simulink model "sm_pump_triplex"  (R2025a)
settings: Solver=VariableStepAuto  StartTime=0.0  StopTime=1.5  RelTol=1e-3  EnableMultiTasking=on
undefined symbols (not defined in the file): pOut_Init_WKSP, smiData, TRP_Par, X, Y, Z
libraries: sm_lib x43, fl_lib x30, nesl_utility x11, simulink x10, SimscapeFluids_lib x3, sm_pump_triplex_lib x3, ee_lib x2, Multibody_Multiphysics_Lib x1
(part 2 of 3)

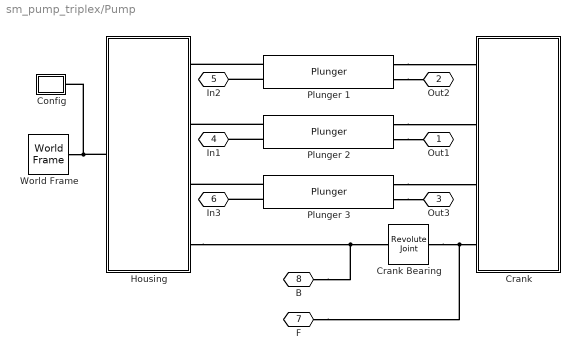
== system sm_pump_triplex/Pump ==
  Config : Subsystem
  Crank : Subsystem  mask(Crankshaft){shaft_len=shaft_len_P, shaft_rad=shaft_rad_P, web_rad=web_rad_P, web_len=web_len_P, motor_shaft_rad=motor_shaft_rad_P, motor_shaft_len=motor_shaft_len_P, shaft_pos=shaft_pos_P, crank_rho=crank_rho_P, motor_shaft_clr=motor_shaft_clr_P, crank_clr=crank_clr_P, crank_opc=crank_opc_P}
      mask prompts: shaft_pos "Crankpin Axis Offset (m)"; crank_rho "Density (kg/m^3)"; motor_shaft_clr "Motor Shaft Color [RGB]"; crank_clr "Crank Color [RGB]"; crank_opc "Opacity (0-1)"
      mask help: Models pump crankshaft with three crankpins, each offset by 120 degrees from the crankshaft axis.
      mask DialogControl text_radius Prompt: Radius (m)
      mask DialogControl text_length Prompt: Length (m)
      mask DialogControl text_crankpin Prompt: Crankpin
      mask DialogControl text_web Prompt: Web
      mask DialogControl text_motor_shaft Prompt: Motor Shaft
      mask DialogControl cont_crank_vis Prompt: Crankshaft Visualization
      mask Display: image('sm_pump_triplex_Crank_IMAGE.png');
  Crank Bearing : sm_lib/Joints/Revolute Joint  JointMode=Normal  CompositeWrenchDir=FollowerOnBase  CompositeWrenchFrame=BaseFrame  SenseConstraintForce=off  SenseConstraintTorque=off  SenseTotalForce=off  SenseTotalTorque=off  PositionTargetSpecify=off  PositionTargetPriority=High  PositionTargetValue=0  PositionTargetValueUnits=deg  VelocityTargetSpecify=off  VelocityTargetPriority=High  VelocityTargetValue=0  VelocityTargetValueUnits=deg/s  EquilibriumPosition=0  EquilibriumPositionUnits=deg  SpringStiffness=0  SpringStiffnessUnits=N*m/deg  DampingCoefficient=bearing_visc_frict  DampingCoefficientUnits=N*m/(deg/s)  LowerLimitSpecify=off  LowerLimitBound=-90  LowerLimitBoundUnits=deg  LowerLimitStiffness=1e4  LowerLimitStiffnessUnits=N*m/deg  LowerLimitDamping=10  LowerLimitDampingUnits=N*m/(deg/s)  LowerLimitTransitionRegionWidth=0.1  LowerLimitTransitionRegionWidthUnits=deg  UpperLimitSpecify=off  UpperLimitBound=90  UpperLimitBoundUnits=deg  UpperLimitStiffness=1e4  UpperLimitStiffnessUnits=N*m/deg  UpperLimitDamping=10  UpperLimitDampingUnits=N*m/(deg/s)  UpperLimitTransitionRegionWidth=0.1  UpperLimitTransitionRegionWidthUnits=deg  TorqueActuationMode=NoTorque  MotionActuationMode=ComputedMotion  SensePosition=off  SenseVelocity=off  SenseAcceleration=off  SenseTorqueForce=off  SenseLowerLimitTorqueForce=off  SenseUpperLimitTorqueForce=off
  Housing : Subsystem
      mask Display: image('sm_pump_triplex_Housing_IMAGE.png');
  Plunger 1 : sm_pump_triplex_lib/Plunger  cyl_gap=cyl_gap_P  cyl_rad_out=cyl_rad_out_P  cyl_len=cyl_len_P  cyl_stroke=cyl_stroke_P  cyl_rad_in=0  cyl_xc_rev=0  cyl_frict_brkway_frc=cyl_frict_brkway_frc_P  cyl_frict_brkway_vel=cyl_frict_brkway_vel_P  cyl_frict_col_frc=cyl_frict_col_frc_P  cyl_frict_visc_coef=cyl_frict_visc_coef_P  cyl_rho=cyl_rho_P  cyl_clr=cyl_clr_P  cyl_opc=cyl_opc_P  plgB_len=plgB_len_P  plgB_rad=plgB_rad_P  stem_len=stem_len_P  stem_rad=stem_rad_P  pin_len=pin_len_P  pin_rad=pin_rad_P  cup_rad_out=cup_rad_out_P  cup_thk=cup_thk_P  cup_len=cup_len_P  cup_pinOffset=cup_pinOffset_P  cup_rad_in=0  plg_rho=plg_rho_P  plg_clr=plg_clr_P  plg_opc=plg_opc_P  conrod_len=conrod_len_P  conrod_web_widP=conrod_web_widP_P  conrod_web_widC=conrod_web_widC_P  conrod_web_offC=0  conrod_web_offP=0  conrod_web_len=0  conrod_web_xc=0  conrod_ringC_wid=conrod_ringC_wid_P  conrod_ringP_wid=conrod_ringP_wid_P  crank_shaft_rad=crank_shaft_rad_P  conrod_ringC_or=0  conrod_ringP_or=0  conrod_ringC_xc_rev=0  conrod_ringP_xc_rev=0  conrod_thk=conrod_thk_P  conrod_rho=conrod_rho_P  conrod_clr=conrod_clr_P  conrod_opc=conrod_opc_P  chkv_in_maxA=chkv_in_maxA_P  chkv_out_maxA=chkv_out_maxA_P  chkv_press_set_popup=Set in Mask  chkv_in_crkP=chkv_in_crkP_P  chkv_out_crkP=chkv_out_crkP_P  chkv_in_maxOpenP=chkv_in_maxOpenP_P  chkv_out_maxOpenP=chkv_out_maxOpenP_P  chkv_vis_popup=On  chkv_vis_rad_in=chkv_vis_rad_in_P  chkv_vis_rad_out=chkv_vis_rad_out_P  chkv_vis_clr_in=chkv_vis_clr_in_P  chkv_vis_clr_out=chkv_vis_clr_out_P  leak_cyl_popup=Off  leak_cyl_area=leak_cyl1_area  block_in_popup=Off  block_in_factor=block_in_cyl1_factor  seal_leak_vis_len=seal_leak_vis_len_P  seal_leak_vis_rad=seal_leak_vis_rad_P  seal_leak_vis_clr=seal_leak_vis_clr_P  seal_leak_vis_opc=0  inlet_obstr_len=inlet_obstr_len_P  inlet_obstr_rad=inlet_obstr_rad_P  inlet_obstr_xc_rev=0  inlet_obstr_clr=inlet_obstr_clr_P  inlet_obstr_opc=1
  Plunger 2 : sm_pump_triplex_lib/Plunger  cyl_gap=cyl_gap_P  cyl_rad_out=cyl_rad_out_P  cyl_len=cyl_len_P  cyl_stroke=cyl_stroke_P  cyl_rad_in=0  cyl_xc_rev=0  cyl_frict_brkway_frc=cyl_frict_brkway_frc_P  cyl_frict_brkway_vel=cyl_frict_brkway_vel_P  cyl_frict_col_frc=cyl_frict_col_frc_P  cyl_frict_visc_coef=cyl_frict_visc_coef_P  cyl_rho=cyl_rho_P  cyl_clr=cyl_clr_P  cyl_opc=cyl_opc_P  plgB_len=plgB_len_P  plgB_rad=plgB_rad_P  stem_len=stem_len_P  stem_rad=stem_rad_P  pin_len=pin_len_P  pin_rad=pin_rad_P  cup_rad_out=cup_rad_out_P  cup_thk=cup_thk_P  cup_len=cup_len_P  cup_pinOffset=cup_pinOffset_P  cup_rad_in=0  plg_rho=plg_rho_P  plg_clr=plg_clr_P  plg_opc=plg_opc_P  conrod_len=conrod_len_P  conrod_web_widP=conrod_web_widP_P  conrod_web_widC=conrod_web_widC_P  conrod_web_offC=0  conrod_web_offP=0  conrod_web_len=0  conrod_web_xc=0  conrod_ringC_wid=conrod_ringC_wid_P  conrod_ringP_wid=conrod_ringP_wid_P  crank_shaft_rad=crank_shaft_rad_P  conrod_ringC_or=0  conrod_ringP_or=0  conrod_ringC_xc_rev=0  conrod_ringP_xc_rev=0  conrod_thk=conrod_thk_P  conrod_rho=conrod_rho_P  conrod_clr=conrod_clr_P  conrod_opc=conrod_opc_P  chkv_in_maxA=chkv_in_maxA_P  chkv_out_maxA=chkv_out_maxA_P  chkv_press_set_popup=Set in Mask  chkv_in_crkP=chkv_in_crkP_P  chkv_out_crkP=chkv_out_crkP_P  chkv_in_maxOpenP=chkv_in_maxOpenP_P  chkv_out_maxOpenP=chkv_out_maxOpenP_P  chkv_vis_popup=On  chkv_vis_rad_in=chkv_vis_rad_in_P  chkv_vis_rad_out=chkv_vis_rad_out_P  chkv_vis_clr_in=chkv_vis_clr_in_P  chkv_vis_clr_out=chkv_vis_clr_out_P  leak_cyl_popup=Off  leak_cyl_area=leak_cyl2_area  block_in_popup=Off  block_in_factor=block_in_cyl2_factor  seal_leak_vis_len=seal_leak_vis_len_P  seal_leak_vis_rad=seal_leak_vis_rad_P  seal_leak_vis_clr=seal_leak_vis_clr_P  seal_leak_vis_opc=0  inlet_obstr_len=inlet_obstr_len_P  inlet_obstr_rad=inlet_obstr_rad_P  inlet_obstr_xc_rev=0  inlet_obstr_clr=inlet_obstr_clr_P  inlet_obstr_opc=1
  Plunger 3 : sm_pump_triplex_lib/Plunger  cyl_gap=cyl_gap_P  cyl_rad_out=cyl_rad_out_P  cyl_len=cyl_len_P  cyl_stroke=cyl_stroke_P  cyl_rad_in=0  cyl_xc_rev=0  cyl_frict_brkway_frc=cyl_frict_brkway_frc_P  cyl_frict_brkway_vel=cyl_frict_brkway_vel_P  cyl_frict_col_frc=cyl_frict_col_frc_P  cyl_frict_visc_coef=cyl_frict_visc_coef_P  cyl_rho=cyl_rho_P  cyl_clr=cyl_clr_P  cyl_opc=cyl_opc_P  plgB_len=plgB_len_P  plgB_rad=plgB_rad_P  stem_len=stem_len_P  stem_rad=stem_rad_P  pin_len=pin_len_P  pin_rad=pin_rad_P  cup_rad_out=cup_rad_out_P  cup_thk=cup_thk_P  cup_len=cup_len_P  cup_pinOffset=cup_pinOffset_P  cup_rad_in=0  plg_rho=plg_rho_P  plg_clr=plg_clr_P  plg_opc=plg_opc_P  conrod_len=conrod_len_P  conrod_web_widP=conrod_web_widP_P  conrod_web_widC=conrod_web_widC_P  conrod_web_offC=0  conrod_web_offP=0  conrod_web_len=0  conrod_web_xc=0  conrod_ringC_wid=conrod_ringC_wid_P  conrod_ringP_wid=conrod_ringP_wid_P  crank_shaft_rad=crank_shaft_rad_P  conrod_ringC_or=0  conrod_ringP_or=0  conrod_ringC_xc_rev=0  conrod_ringP_xc_rev=0  conrod_thk=conrod_thk_P  conrod_rho=conrod_rho_P  conrod_clr=conrod_clr_P  conrod_opc=conrod_opc_P  chkv_in_maxA=chkv_in_maxA_P  chkv_out_maxA=chkv_out_maxA_P  chkv_press_set_popup=Set in Mask  chkv_in_crkP=chkv_in_crkP_P  chkv_out_crkP=chkv_out_crkP_P  chkv_in_maxOpenP=chkv_in_maxOpenP_P  chkv_out_maxOpenP=chkv_out_maxOpenP_P  chkv_vis_popup=On  chkv_vis_rad_in=chkv_vis_rad_in_P  chkv_vis_rad_out=chkv_vis_rad_out_P  chkv_vis_clr_in=chkv_vis_clr_in_P  chkv_vis_clr_out=chkv_vis_clr_out_P  leak_cyl_popup=Off  leak_cyl_area=leak_cyl3_area  block_in_popup=Off  block_in_factor=block_in_cyl3_factor  seal_leak_vis_len=seal_leak_vis_len_P  seal_leak_vis_rad=seal_leak_vis_rad_P  seal_leak_vis_clr=seal_leak_vis_clr_P  seal_leak_vis_opc=0  inlet_obstr_len=inlet_obstr_len_P  inlet_obstr_rad=inlet_obstr_rad_P  inlet_obstr_xc_rev=0  inlet_obstr_clr=inlet_obstr_clr_P  inlet_obstr_opc=1
  World Frame : sm_lib/Frames and Transforms/World Frame
  Out1 : PMIOPort  Side=Right
  Out2 : PMIOPort  Port=2  Side=Right
  Out3 : PMIOPort  Port=3  Side=Right
  In1 : PMIOPort  Port=4  Side=Right
  In2 : PMIOPort  Port=5  Side=Right
  In3 : PMIOPort  Port=6  Side=Right
  F : PMIOPort  Port=7  Side=Left
  B : PMIOPort  Port=8  Side=Left
  connections:
  Housing/LConn1 -- World Frame/RConn1 -- Config/RConn1
  Plunger 2/LConn1 -- Housing/RConn2
  Plunger 1/LConn2 -- In2/RConn1
  Plunger 1/RConn1 -- Crank/LConn1
  Plunger 2/RConn1 -- Crank/LConn2
  Plunger 3/LConn2 -- In3/RConn1
  Plunger 3/RConn2 -- Out3/RConn1
  Plunger 1/LConn1 -- Housing/RConn1
  Plunger 2/LConn2 -- In1/RConn1
  Plunger 3/LConn1 -- Housing/RConn3
  Housing/RConn4 -- B/RConn1 -- Crank Bearing/LConn1
  Crank Bearing/RConn1 -- F/RConn1 -- Crank/LConn4
  Plunger 1/RConn2 -- Out2/RConn1
  Plunger 2/RConn2 -- Out1/RConn1
  Plunger 3/RConn1 -- Crank/LConn3

== system sm_pump_triplex/Sensing Current ==
  Current Sensor : fl_lib/Electrical/Electrical Sensors/Current Sensor
  Current with Noise : Scope  NumInputPorts=2
      settings: ActiveDisplayYMinimum=-5.56656  ActiveDisplayYMaximum=49.76256  DataLoggingVariableName=ScopeData2
  Measurement Noise : simulink/Sources/Band-Limited White Noise  Cov=TRP_Par.Sensors.i.Np  Ts=TRP_Par.Sensors.i.Ts  seed=[23345]
  PS-Simulink Converter : nesl_utility/PS-Simulink Converter  PhysicalDomain=network_engine_domain  SubClassName=ps_output  LeftPortType=input  RightPortType=output  PseudoPeriodic=off  Frequencies=[]  VectorFormat=1-D array  Unit=1  AffineConversion=off
  Sum1 : Sum  Inputs=++|
  Zero-Order Hold : ZeroOrderHold  SampleTime=TRP_Par.Sensors.i.Ts
  - : PMIOPort  Side=Right
  + : PMIOPort  Port=2  Side=Left
  wires:
  Measurement Noise/1 -> Sum1/1  "Noise"
  Sum1/1 -> Zero-Order Hold/1
  PS-Simulink Converter/1 -> Sum1/2, Current with Noise/2
  Zero-Order Hold/1 -> Current with Noise/1
  connections:
  PS-Simulink Converter/LConn1 -- Current Sensor/RConn1
  +/RConn1 -- Current Sensor/LConn1
  Current Sensor/RConn2 -- -/RConn1

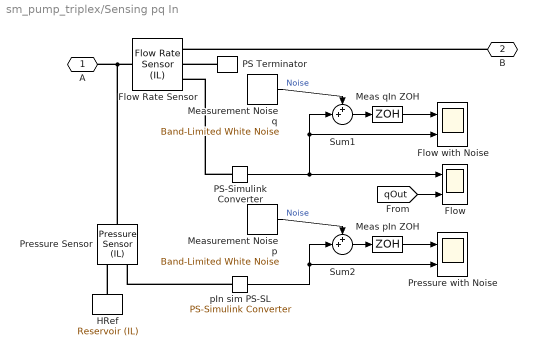
== system sm_pump_triplex/Sensing pq In ==
  Flow : Scope  NumInputPorts=2
      settings: ActiveDisplayYMinimum=-6.56594  ActiveDisplayYMaximum=59.09339  DataLoggingVariableName=ScopeData2
  Flow Rate Sensor : fl_lib/Isothermal Liquid/Sensors/Flow Rate Sensor (IL)  sensor_type=3
      settings: InternalSimscapePortConfiguration="{\"Bottom\":[],\"Left\":[{\"id\":\"A\",\"label\":\"A\",\"type\":\"foundation.isothermal_liquid.isothermal_liquid\"}],\"Right\":[{\"id\":\"B\",\"label\":\"B\",\"type\":\"foundation.isothermal_liquid.isothermal_liquid\"},{\"id\":\"M\",\"label\":\"M\",\"type\":\"output\"},{\"id\":\"V\",\"label\":\"V\",\"type\":\"output\"}],\"Top\":[]}"
      settings: LibrarySourceBlock=|
      | fl_lib/Hydraulic/Hydraulic Sensors/Hydraulic Flow Rate
      | Sensor
  Flow with Noise : Scope  NumInputPorts=2
      settings: ActiveDisplayYMinimum=-7.18648  ActiveDisplayYMaximum=60.19336
  HRef : fl_lib/Isothermal Liquid/Elements/Reservoir (IL)  reservoir_type=foundation.enum.constant_controlled.constant  pressure_spec=foundation.enum.pressure_spec.atmospheric  reservoir_pressure=0.101325 MPa
      settings: LibrarySourceBlock=fl_lib/Hydraulic/Hydraulic Elements/Hydraulic Reference
  Meas pIn ZOH : ZeroOrderHold  SampleTime=TRP_Par.Sensors.p.Ts
  Meas qIn ZOH : ZeroOrderHold  SampleTime=TRP_Par.Sensors.q.Ts
  Measurement Noise p : simulink/Sources/Band-Limited White Noise  Cov=TRP_Par.Sensors.p.Np  Ts=TRP_Par.Sensors.p.Ts  seed=[23345]
  Measurement Noise q : simulink/Sources/Band-Limited White Noise  Cov=TRP_Par.Sensors.q.Np  Ts=TRP_Par.Sensors.q.Ts  seed=[23345]
  PS Terminator : fl_lib/Physical Signals/Sinks/PS Terminator
  PS-Simulink Converter : nesl_utility/PS-Simulink Converter  PhysicalDomain=network_engine_domain  SubClassName=ps_output  LeftPortType=input  RightPortType=output  PseudoPeriodic=off  Frequencies=[]  VectorFormat=1-D array  Unit=lpm  AffineConversion=off
  Pressure Sensor : fl_lib/Isothermal Liquid/Sensors/Pressure Sensor (IL)  pressure_measure=foundation.enum.pressure_measure.difference
      settings: InternalSimscapePortConfiguration="{\"Bottom\":[],\"Left\":[{\"id\":\"A\",\"label\":\"A\",\"type\":\"foundation.isothermal_liquid.isothermal_liquid\"}],\"Right\":[{\"id\":\"B\",\"label\":\"B\",\"type\":\"foundation.isothermal_liquid.isothermal_liquid\"},{\"id\":\"P\",\"label\":\"P\",\"type\":\"output\"}],\"Top\":[]}"
      settings: LibrarySourceBlock=|
      | fl_lib/Hydraulic/Hydraulic Sensors/Hydraulic Pressure
      | Sensor
  Pressure with Noise : Scope  NumInputPorts=2
      settings: ActiveDisplayYMinimum=6.95483  ActiveDisplayYMaximum=7.36166
  Sum1 : Sum  Inputs=++|
  Sum2 : Sum  Inputs=++|
  pIn sim PS-SL : nesl_utility/PS-Simulink Converter  PhysicalDomain=network_engine_domain  SubClassName=ps_output  LeftPortType=input  RightPortType=output  PseudoPeriodic=off  Frequencies=[]  VectorFormat=1-D array  Unit=bar  AffineConversion=off
  A : PMIOPort  Side=Left
  B : PMIOPort  Port=2  Side=Right
  wires:
  Meas pIn ZOH/1 -> Pressure with Noise/1
  Measurement Noise p/1 -> Sum2/1  "Noise"
  pIn sim PS-SL/1 -> Pressure with Noise/2, Sum2/2
  Sum2/1 -> Meas pIn ZOH/1
  Meas qIn ZOH/1 -> Flow with Noise/1
  Sum1/1 -> Meas qIn ZOH/1
  Measurement Noise q/1 -> Sum1/1  "Noise"
  PS-Simulink Converter/1 -> Flow/1, Flow with Noise/2, Sum1/2
  [qOut] -> Flow/2
  connections:
  pIn sim PS-SL/LConn1 -- Pressure Sensor/RConn2
  HRef/LConn1 -- Pressure Sensor/RConn1
  Pressure Sensor/LConn1 -- Flow Rate Sensor/LConn1 -- A/RConn1
  PS Terminator/LConn1 -- Flow Rate Sensor/RConn2
  B/RConn1 -- Flow Rate Sensor/RConn1
  PS-Simulink Converter/LConn1 -- Flow Rate Sensor/RConn3

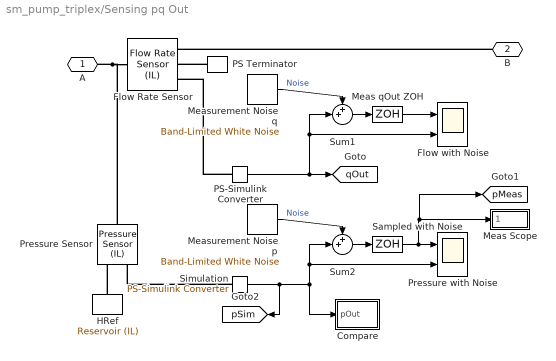
== system sm_pump_triplex/Sensing pq Out ==
  Compare : Subsystem
  Flow Rate Sensor : fl_lib/Isothermal Liquid/Sensors/Flow Rate Sensor (IL)  sensor_type=3
      settings: InternalSimscapePortConfiguration="{\"Bottom\":[],\"Left\":[{\"id\":\"A\",\"label\":\"A\",\"type\":\"foundation.isothermal_liquid.isothermal_liquid\"}],\"Right\":[{\"id\":\"B\",\"label\":\"B\",\"type\":\"foundation.isothermal_liquid.isothermal_liquid\"},{\"id\":\"M\",\"label\":\"M\",\"type\":\"output\"},{\"id\":\"V\",\"label\":\"V\",\"type\":\"output\"}],\"Top\":[]}"
      settings: LibrarySourceBlock=|
      | fl_lib/Hydraulic/Hydraulic Sensors/Hydraulic Flow Rate
      | Sensor
  Flow with Noise : Scope  NumInputPorts=2
      settings: ActiveDisplayYMinimum=-6.25341  ActiveDisplayYMaximum=51.79569
  HRef : fl_lib/Isothermal Liquid/Elements/Reservoir (IL)  reservoir_type=foundation.enum.constant_controlled.constant  pressure_spec=foundation.enum.pressure_spec.atmospheric  reservoir_pressure=0.101325 MPa
      settings: LibrarySourceBlock=fl_lib/Hydraulic/Hydraulic Elements/Hydraulic Reference
  Meas Scope : Subsystem
  Meas qOut ZOH : ZeroOrderHold  SampleTime=TRP_Par.Sensors.q.Ts
  Measurement Noise p : simulink/Sources/Band-Limited White Noise  Cov=TRP_Par.Sensors.p.Np  Ts=TRP_Par.Sensors.p.Ts  seed=[23345]
  Measurement Noise q : simulink/Sources/Band-Limited White Noise  Cov=TRP_Par.Sensors.q.Np  Ts=TRP_Par.Sensors.q.Ts  seed=[23345]
  PS Terminator : fl_lib/Physical Signals/Sinks/PS Terminator
  PS-Simulink Converter : nesl_utility/PS-Simulink Converter  PhysicalDomain=network_engine_domain  SubClassName=ps_output  LeftPortType=input  RightPortType=output  PseudoPeriodic=off  Frequencies=[]  VectorFormat=1-D array  Unit=lpm  AffineConversion=off
  Pressure Sensor : fl_lib/Isothermal Liquid/Sensors/Pressure Sensor (IL)  pressure_measure=foundation.enum.pressure_measure.difference
      settings: InternalSimscapePortConfiguration="{\"Bottom\":[],\"Left\":[{\"id\":\"A\",\"label\":\"A\",\"type\":\"foundation.isothermal_liquid.isothermal_liquid\"}],\"Right\":[{\"id\":\"B\",\"label\":\"B\",\"type\":\"foundation.isothermal_liquid.isothermal_liquid\"},{\"id\":\"P\",\"label\":\"P\",\"type\":\"output\"}],\"Top\":[]}"
      settings: LibrarySourceBlock=|
      | fl_lib/Hydraulic/Hydraulic Sensors/Hydraulic Pressure
      | Sensor
  Pressure with Noise : Scope  NumInputPorts=2
      settings: ActiveDisplayYMinimum=6.95483  ActiveDisplayYMaximum=7.36166
  Sampled with Noise : ZeroOrderHold  SampleTime=TRP_Par.Sensors.p.Ts
  Simulation : nesl_utility/PS-Simulink Converter  PhysicalDomain=network_engine_domain  SubClassName=ps_output  LeftPortType=input  RightPortType=output  PseudoPeriodic=off  Frequencies=[]  VectorFormat=1-D array  Unit=bar  AffineConversion=off
  Sum1 : Sum  Inputs=++|
  Sum2 : Sum  Inputs=++|
  A : PMIOPort  Side=Left
  B : PMIOPort  Port=2  Side=Right
  tag scope: pMeas=global, pSim=global, qOut=global
  wires:
  PS-Simulink Converter/1 -> Sum1/2, Flow with Noise/2, [qOut]
  Measurement Noise q/1 -> Sum1/1  "Noise"
  Sum1/1 -> Meas qOut ZOH/1
  Meas qOut ZOH/1 -> Flow with Noise/1
  Sum2/1 -> Sampled with Noise/1
  Simulation/1 -> [pSim], Compare/1(pOut), Sum2/2, Pressure with Noise/2
  Measurement Noise p/1 -> Sum2/1  "Noise"
  Sampled with Noise/1 -> [pMeas], Meas Scope/1(pMeas), Pressure with Noise/1
  connections:
  Pressure Sensor/LConn1 -- Flow Rate Sensor/LConn1 -- A/RConn1
  HRef/LConn1 -- Pressure Sensor/RConn1
  Simulation/LConn1 -- Pressure Sensor/RConn2
  PS Terminator/LConn1 -- Flow Rate Sensor/RConn2
  B/RConn1 -- Flow Rate Sensor/RConn1
  PS-Simulink Converter/LConn1 -- Flow Rate Sensor/RConn3

== system sm_pump_triplex/Diagnostics/Diagnostics ==
  "pOut " : Inport
  Off : Subsystem  VariantControl=Off
  On : Subsystem  VariantControl=On
  " fault" : Outport  VectorParamsAs1DForOutWhenUnconnected=off
  " hmi" : Outport  Port=2  VectorParamsAs1DForOutWhenUnconnected=off

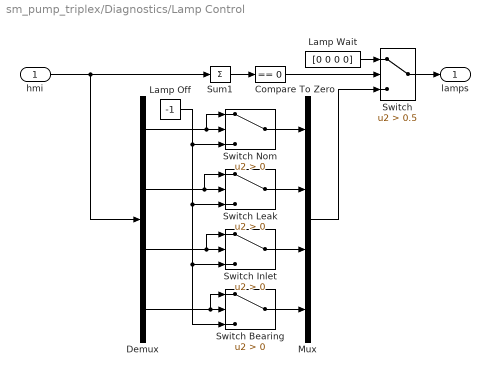
== system sm_pump_triplex/Diagnostics/Lamp Control ==
  hmi : Inport
  Compare To Zero : simulink/Logic and Bit Operations/Compare To Zero  relop===  OutDataTypeStr=boolean  ZeroCross=off
  Demux : Demux
  Lamp Off : Constant  Value=-1
  Lamp Wait : Constant  Value=[0 0 0 0]
  Mux : Mux
  Sum1 : Sum  Inputs=+
  Switch : Switch  Criteria=u2 > Threshold  Threshold=0.5  ZeroCross=off  SaturateOnIntegerOverflow=off  InputSameDT=off
  Switch Bearing : Switch  Criteria=u2 > Threshold  ZeroCross=off  SaturateOnIntegerOverflow=off  InputSameDT=off
  Switch Inlet : Switch  Criteria=u2 > Threshold  ZeroCross=off  SaturateOnIntegerOverflow=off  InputSameDT=off
  Switch Leak : Switch  Criteria=u2 > Threshold  ZeroCross=off  SaturateOnIntegerOverflow=off  InputSameDT=off
  Switch Nom : Switch  Criteria=u2 > Threshold  ZeroCross=off  SaturateOnIntegerOverflow=off  InputSameDT=off
  lamps : Outport  VectorParamsAs1DForOutWhenUnconnected=off
  wires:
  Compare To Zero/1 -> Switch/2
  Sum1/1 -> Compare To Zero/1
  hmi/1 -> Demux/1, Sum1/1
  Switch/1 -> lamps/1
  Lamp Wait/1 -> Switch/1
  Switch Nom/1 -> Mux/1
  Switch Leak/1 -> Mux/2
  Switch Inlet/1 -> Mux/3
  Switch Bearing/1 -> Mux/4
  Mux/1 -> Switch/3
  Demux/1 -> Switch Nom/1, Switch Nom/2
  Demux/2 -> Switch Leak/1, Switch Leak/2
  Demux/3 -> Switch Inlet/1, Switch Inlet/2
  Demux/4 -> Switch Bearing/1, Switch Bearing/2
  Lamp Off/1 -> Switch Bearing/3, Switch Inlet/3, Switch Leak/3, Switch Nom/3

== system sm_pump_triplex/Driver/Driver ==
  Dyno : Subsystem  VariantControl=Dyno
      mask Display: image('sm_pump_triplex_driverDyno_IMAGE.png');
  Motor : Subsystem  VariantControl=Motor  mask{winding_fault_enable=Off, winding_fault_sw=0}
      mask prompts: winding_fault_enable "Winding Fault"; winding_fault_sw "Winding Fault Input for Switch (1,2)"
      mask init:
      | if(strcmp(get_param(gcb,'winding_fault_enable'),'Off'))
      |     winding_fault_sw = 1;
      | else
      |     winding_fault_sw = 2;
      | end
      mask TypeOptions winding_fault_enable: Off | On
      mask Display:
      | image('sm_pump_triplex_driverMotor_IMAGE.png');
      | 
      | color('red');
      | if(strcmp(get_param(gcb,'winding_fault_enable'),'On'))
      |     plot([0.85 0.6],[1.1 0.9])
      |     plot([0.6 0.85],[1.1 0.9])
      | end
      | 
      | % Plot points to set plot range
      | color('white');plot(1.2,2.4);plot(-1.2,-2.4)
      | color('black');
  " F " : PMIOPort  Side=Right
  " B " : PMIOPort  Port=2  Side=Right
  " + " : PMIOPort  Port=3  Side=Left
  " - " : PMIOPort  Port=4  Side=Left

== system sm_pump_triplex/Pump/Config ==
  Mechanism Configuration : sm_lib/Utilities/Mechanism Configuration  UniformGravity=Constant  GravityVector=[0 -1 0]*9.80665  GravityVectorUnits=m/s^2  LinearizationDelta=0.001  JointModeTransitionNonlinearIterations=2
  Solver Configuration : nesl_utility/Solver Configuration  PhysicalDomain=network_engine_domain  SubClassName=solver  LeftPortType=input  RightPortType=generic  Tones=[]  Harmonics=[]  SimulateNoise=off  Profile=off  UseLocalSampling=off  EnableSwitchedLinearOptims=on  FrequencyDomain=off  UseCCode=off  RelTol=0.001  AbsTol=1e-06  MinStep=1e-09  ToWorkspace=off  RevertToSquareIcSolve=off  NumHomotopyIterations=100  PhasorMode=off  PhasorModeNumHarmonics=1  ConsistencySolver=NEWTON_FTOL  IndexReductionMethod=DerivativeReplacement  DoDC=off  ResidualTolerance=1e-10  ConsistencyTolSource=GLOBAL  ConsistencyAbsTol=0.001  ConsistencyRelTol=0.001  ConsistencyTolFactor=0.001  UseLocalSolver=off  LocalSolverChoice=NE_BACKWARD_EULER_ADVANCER  ResolveIndetEquations=on  FunctionEvalNumThread=1  LocalSolverSampleTime=0.001  DoFixedCost=off  MaxNonlinIter=3  MaxModeIter=2  ComputeImpulses=off  ImpulseIterations=2  LinearAlgebra=Sparse  LinearAlgebraNumThread=0  EquationFormulation=NE_TIME_EF  DelaysMemoryBudget=1024  AutomaticFiltering=on  FilteringTimeConstant=0.001  PartitionStorageMethod=AS_NEEDED  PartitionMemoryBudget=1024  PartitionMethod=FAST  MultibodyUseLocalSolver=off  MultibodyLocalSolverChoice=ODE1  MultibodyLocalSolverSampleTime=0.001
  C : PMIOPort  Side=Right
  connections:
  Solver Configuration/RConn1 -- C/RConn1 -- Mechanism Configuration/RConn1

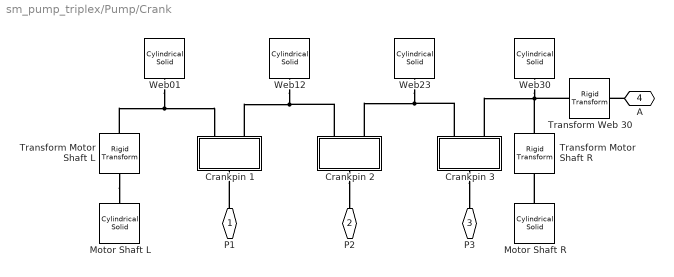
== system sm_pump_triplex/Pump/Crank ==
  Crankpin 1 : Subsystem
  Crankpin 2 : Subsystem
  Crankpin 3 : Subsystem
  Motor Shaft L : sm_lib/Body Elements/Cylindrical Solid  CylinderRadius=motor_shaft_rad  CylinderRadiusUnits=m  CylinderLength=motor_shaft_len  CylinderLengthUnits=m  ExportEntireGeometry=off  InertiaType=CalculateFromGeometry  BasedOnType=Density  Density=crank_rho  DensityUnits=kg/m^3  Mass=1  MassUnits=kg  CenterOfMass=[0 0 0]  CenterOfMassUnits=m  MomentsOfInertia=[1 1 1]  MomentsOfInertiaUnits=kg*m^2  ProductsOfInertia=[1 1 1]  ProductsOfInertiaUnits=kg*m^2  GraphicType=FromGeometry  MarkerShape=Sphere  MarkerSize=10  GraphicVisPropType=SimpleVisualProperties  GraphicDiffuseColor=motor_shaft_clr  GraphicOpacity=crank_opc  GraphicSpecularColor=[0.5 0.5 0.5 1.0]  GraphicAmbientColor=[0.15 0.15 0.15 1.0]  GraphicEmissiveColor=[0.0 0.0 0.0 1.0]  GraphicShininess=75  DoExposeReferenceFrame=on  SerializedFrames=<Frames/>
  Motor Shaft R : sm_lib/Body Elements/Cylindrical Solid  CylinderRadius=motor_shaft_rad  CylinderRadiusUnits=m  CylinderLength=motor_shaft_len  CylinderLengthUnits=m  ExportEntireGeometry=off  InertiaType=CalculateFromGeometry  BasedOnType=Density  Density=crank_rho  DensityUnits=kg/m^3  Mass=1  MassUnits=kg  CenterOfMass=[0 0 0]  CenterOfMassUnits=m  MomentsOfInertia=[1 1 1]  MomentsOfInertiaUnits=kg*m^2  ProductsOfInertia=[1 1 1]  ProductsOfInertiaUnits=kg*m^2  GraphicType=FromGeometry  MarkerShape=Sphere  MarkerSize=10  GraphicVisPropType=SimpleVisualProperties  GraphicDiffuseColor=motor_shaft_clr  GraphicOpacity=crank_opc  GraphicSpecularColor=[0.5 0.5 0.5 1.0]  GraphicAmbientColor=[0.15 0.15 0.15 1.0]  GraphicEmissiveColor=[0.0 0.0 0.0 1.0]  GraphicShininess=75  DoExposeReferenceFrame=on  SerializedFrames=<Frames/>
  Transform Motor Shaft L : sm_lib/Frames and Transforms/Rigid Transform  RotationMethod=None  FollAlignAxisA=+X  BaseAlignAxisA=+Y  FollAlignAxisB=+Y  BaseAlignAxisB=+Z  RotationStandardAxis=+Z  RotationAngle=0.0  RotationAngleUnits=deg  RotationArbitraryAxis=[0 0 1]  RotationSequenceAxes=FollowerAxes  RotationSequence=XYX  RotationSequenceAngles=[0 0 0]  RotationSequenceAnglesUnits=deg  RotationMatrix=[1 0 0; 0 1 0; 0 0 1]  Quaternion=[1 0 0 0]  TranslationMethod=StandardAxis  TranslationCartesianOffset=[0 0 0]  TranslationCartesianOffsetUnits=m  TranslationStandardAxis=+Z  TranslationStandardOffset=motor_shaft_len/2  TranslationStandardOffsetUnits=m  TranslationROffset=0  TranslationROffsetUnits=m  TranslationThetaOffset=0  TranslationThetaOffsetUnits=deg  TranslationZOffset=0  TranslationZOffsetUnits=m
  Transform Motor Shaft R : sm_lib/Frames and Transforms/Rigid Transform  RotationMethod=None  FollAlignAxisA=+X  BaseAlignAxisA=+Y  FollAlignAxisB=+Y  BaseAlignAxisB=+Z  RotationStandardAxis=+Z  RotationAngle=0.0  RotationAngleUnits=deg  RotationArbitraryAxis=[0 0 1]  RotationSequenceAxes=FollowerAxes  RotationSequence=XYX  RotationSequenceAngles=[0 0 0]  RotationSequenceAnglesUnits=deg  RotationMatrix=[1 0 0; 0 1 0; 0 0 1]  Quaternion=[1 0 0 0]  TranslationMethod=StandardAxis  TranslationCartesianOffset=[0 0 0]  TranslationCartesianOffsetUnits=m  TranslationStandardAxis=+Z  TranslationStandardOffset=motor_shaft_len/2  TranslationStandardOffsetUnits=m  TranslationROffset=0  TranslationROffsetUnits=m  TranslationThetaOffset=0  TranslationThetaOffsetUnits=deg  TranslationZOffset=0  TranslationZOffsetUnits=m
  Transform Web 30 : sm_lib/Frames and Transforms/Rigid Transform  RotationMethod=None  FollAlignAxisA=+X  BaseAlignAxisA=+Y  FollAlignAxisB=+Y  BaseAlignAxisB=+Z  RotationStandardAxis=+Z  RotationAngle=0.0  RotationAngleUnits=deg  RotationArbitraryAxis=[0 0 1]  RotationSequenceAxes=FollowerAxes  RotationSequence=XYX  RotationSequenceAngles=[0 0 0]  RotationSequenceAnglesUnits=deg  RotationMatrix=[1 0 0; 0 1 0; 0 0 1]  Quaternion=[1 0 0 0]  TranslationMethod=StandardAxis  TranslationCartesianOffset=[0 0 0]  TranslationCartesianOffsetUnits=m  TranslationStandardAxis=+Z  TranslationStandardOffset=shaft_len*1.5  TranslationStandardOffsetUnits=m  TranslationROffset=0  TranslationROffsetUnits=m  TranslationThetaOffset=0  TranslationThetaOffsetUnits=deg  TranslationZOffset=0  TranslationZOffsetUnits=m
  Web01 : sm_lib/Body Elements/Cylindrical Solid  CylinderRadius=web_rad  CylinderRadiusUnits=m  CylinderLength=web_len  CylinderLengthUnits=m  ExportEntireGeometry=off  InertiaType=CalculateFromGeometry  BasedOnType=Density  Density=crank_rho  DensityUnits=kg/m^3  Mass=1  MassUnits=kg  CenterOfMass=[0 0 0]  CenterOfMassUnits=m  MomentsOfInertia=[1 1 1]  MomentsOfInertiaUnits=kg*m^2  ProductsOfInertia=[1 1 1]  ProductsOfInertiaUnits=kg*m^2  GraphicType=FromGeometry  MarkerShape=Sphere  MarkerSize=10  GraphicVisPropType=SimpleVisualProperties  GraphicDiffuseColor=crank_clr  GraphicOpacity=crank_opc  GraphicSpecularColor=[0.5 0.5 0.5 1.0]  GraphicAmbientColor=[0.15 0.15 0.15 1.0]  GraphicEmissiveColor=[0.0 0.0 0.0 1.0]  GraphicShininess=75  DoExposeReferenceFrame=on  SerializedFrames=<Frames/>
  Web12 : sm_lib/Body Elements/Cylindrical Solid  CylinderRadius=web_rad  CylinderRadiusUnits=m  CylinderLength=web_len  CylinderLengthUnits=m  ExportEntireGeometry=off  InertiaType=CalculateFromGeometry  BasedOnType=Density  Density=crank_rho  DensityUnits=kg/m^3  Mass=1  MassUnits=kg  CenterOfMass=[0 0 0]  CenterOfMassUnits=m  MomentsOfInertia=[1 1 1]  MomentsOfInertiaUnits=kg*m^2  ProductsOfInertia=[1 1 1]  ProductsOfInertiaUnits=kg*m^2  GraphicType=FromGeometry  MarkerShape=Sphere  MarkerSize=10  GraphicVisPropType=SimpleVisualProperties  GraphicDiffuseColor=crank_clr  GraphicOpacity=crank_opc  GraphicSpecularColor=[0.5 0.5 0.5 1.0]  GraphicAmbientColor=[0.15 0.15 0.15 1.0]  GraphicEmissiveColor=[0.0 0.0 0.0 1.0]  GraphicShininess=75  DoExposeReferenceFrame=on  SerializedFrames=<Frames/>
  Web23 : sm_lib/Body Elements/Cylindrical Solid  CylinderRadius=web_rad  CylinderRadiusUnits=m  CylinderLength=web_len  CylinderLengthUnits=m  ExportEntireGeometry=off  InertiaType=CalculateFromGeometry  BasedOnType=Density  Density=crank_rho  DensityUnits=kg/m^3  Mass=1  MassUnits=kg  CenterOfMass=[0 0 0]  CenterOfMassUnits=m  MomentsOfInertia=[1 1 1]  MomentsOfInertiaUnits=kg*m^2  ProductsOfInertia=[1 1 1]  ProductsOfInertiaUnits=kg*m^2  GraphicType=FromGeometry  MarkerShape=Sphere  MarkerSize=10  GraphicVisPropType=SimpleVisualProperties  GraphicDiffuseColor=crank_clr  GraphicOpacity=crank_opc  GraphicSpecularColor=[0.5 0.5 0.5 1.0]  GraphicAmbientColor=[0.15 0.15 0.15 1.0]  GraphicEmissiveColor=[0.0 0.0 0.0 1.0]  GraphicShininess=75  DoExposeReferenceFrame=on  SerializedFrames=<Frames/>
  Web30 : sm_lib/Body Elements/Cylindrical Solid  CylinderRadius=web_rad  CylinderRadiusUnits=m  CylinderLength=web_len  CylinderLengthUnits=m  ExportEntireGeometry=off  InertiaType=CalculateFromGeometry  BasedOnType=Density  Density=crank_rho  DensityUnits=kg/m^3  Mass=1  MassUnits=kg  CenterOfMass=[0 0 0]  CenterOfMassUnits=m  MomentsOfInertia=[1 1 1]  MomentsOfInertiaUnits=kg*m^2  ProductsOfInertia=[1 1 1]  ProductsOfInertiaUnits=kg*m^2  GraphicType=FromGeometry  MarkerShape=Sphere  MarkerSize=10  GraphicVisPropType=SimpleVisualProperties  GraphicDiffuseColor=crank_clr  GraphicOpacity=crank_opc  GraphicSpecularColor=[0.5 0.5 0.5 1.0]  GraphicAmbientColor=[0.15 0.15 0.15 1.0]  GraphicEmissiveColor=[0.0 0.0 0.0 1.0]  GraphicShininess=75  DoExposeReferenceFrame=on  SerializedFrames=<Frames/>
  P1 : PMIOPort  Side=Left
  P2 : PMIOPort  Port=2  Side=Left
  P3 : PMIOPort  Port=3  Side=Left
  A : PMIOPort  Port=4  Side=Left
  connections:
  Crankpin 2/LConn2 -- Web23/RConn1 -- Crankpin 3/LConn1
  Motor Shaft R/RConn1 -- Transform Motor Shaft R/RConn1
  Crankpin 1/LConn2 -- Web12/RConn1 -- Crankpin 2/LConn1
  Crankpin 2/RConn1 -- P2/RConn1
  Web01/RConn1 -- Transform Motor Shaft L/RConn1 -- Crankpin 1/LConn1
  P1/RConn1 -- Crankpin 1/RConn1
  Crankpin 3/RConn1 -- P3/RConn1
  Transform Motor Shaft R/LConn1 -- Transform Web 30/RConn1 -- Web30/RConn1 -- Crankpin 3/LConn2
  Transform Motor Shaft L/LConn1 -- Motor Shaft L/RConn1
  A/RConn1 -- Transform Web 30/LConn1

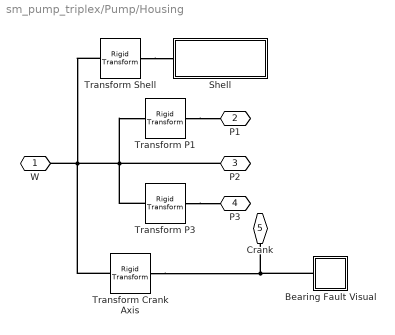
== system sm_pump_triplex/Pump/Housing ==
  Bearing Fault Visual : Subsystem
  Shell : Subsystem
  Transform Crank Axis : sm_lib/Frames and Transforms/Rigid Transform  RotationMethod=StandardAxis  FollAlignAxisA=+X  BaseAlignAxisA=+Y  FollAlignAxisB=+Y  BaseAlignAxisB=+Z  RotationStandardAxis=+Y  RotationAngle=90  RotationAngleUnits=deg  RotationArbitraryAxis=[0 0 1]  RotationSequenceAxes=FollowerAxes  RotationSequence=XYX  RotationSequenceAngles=[0 0 0]  RotationSequenceAnglesUnits=deg  RotationMatrix=[1 0 0; 0 1 0; 0 0 1]  Quaternion=[1 0 0 0]  TranslationMethod=Cartesian  TranslationCartesianOffset=crank_ax_offset  TranslationCartesianOffsetUnits=m  TranslationStandardAxis=+Z  TranslationStandardOffset=0  TranslationStandardOffsetUnits=m  TranslationROffset=0  TranslationROffsetUnits=m  TranslationThetaOffset=0  TranslationThetaOffsetUnits=deg  TranslationZOffset=0  TranslationZOffsetUnits=m
  Transform Shell : sm_lib/Frames and Transforms/Rigid Transform  RotationMethod=StandardAxis  FollAlignAxisA=+X  BaseAlignAxisA=+Y  FollAlignAxisB=+Y  BaseAlignAxisB=+Z  RotationStandardAxis=+Y  RotationAngle=180  RotationAngleUnits=deg  RotationArbitraryAxis=[0 0 1]  RotationSequenceAxes=FollowerAxes  RotationSequence=XYX  RotationSequenceAngles=[0 0 0]  RotationSequenceAnglesUnits=deg  RotationMatrix=[1 0 0; 0 1 0; 0 0 1]  Quaternion=[1 0 0 0]  TranslationMethod=Cartesian  TranslationCartesianOffset=TRP_Par.CAD.offset  TranslationCartesianOffsetUnits=m  TranslationStandardAxis=+Z  TranslationStandardOffset=0  TranslationStandardOffsetUnits=m  TranslationROffset=0  TranslationROffsetUnits=m  TranslationThetaOffset=0  TranslationThetaOffsetUnits=deg  TranslationZOffset=0  TranslationZOffsetUnits=m
  Transform P1 : sm_lib/Frames and Transforms/Rigid Transform  RotationMethod=None  FollAlignAxisA=+X  BaseAlignAxisA=+Y  FollAlignAxisB=+Y  BaseAlignAxisB=+Z  RotationStandardAxis=+Z  RotationAngle=0.0  RotationAngleUnits=deg  RotationArbitraryAxis=[0 0 1]  RotationSequenceAxes=FollowerAxes  RotationSequence=XYX  RotationSequenceAngles=[0 0 0]  RotationSequenceAnglesUnits=deg  RotationMatrix=[1 0 0; 0 1 0; 0 0 1]  Quaternion=[1 0 0 0]  TranslationMethod=StandardAxis  TranslationCartesianOffset=[0 0 0]  TranslationCartesianOffsetUnits=m  TranslationStandardAxis=+X  TranslationStandardOffset=-TRP_Par.Crank.Shaft.len  TranslationStandardOffsetUnits=m  TranslationROffset=0  TranslationROffsetUnits=m  TranslationThetaOffset=0  TranslationThetaOffsetUnits=deg  TranslationZOffset=0  TranslationZOffsetUnits=m
  Transform P3 : sm_lib/Frames and Transforms/Rigid Transform  RotationMethod=None  FollAlignAxisA=+X  BaseAlignAxisA=+Y  FollAlignAxisB=+Y  BaseAlignAxisB=+Z  RotationStandardAxis=+Z  RotationAngle=0.0  RotationAngleUnits=deg  RotationArbitraryAxis=[0 0 1]  RotationSequenceAxes=FollowerAxes  RotationSequence=XYX  RotationSequenceAngles=[0 0 0]  RotationSequenceAnglesUnits=deg  RotationMatrix=[1 0 0; 0 1 0; 0 0 1]  Quaternion=[1 0 0 0]  TranslationMethod=StandardAxis  TranslationCartesianOffset=[0 0 0]  TranslationCartesianOffsetUnits=m  TranslationStandardAxis=-X  TranslationStandardOffset=-TRP_Par.Crank.Shaft.len  TranslationStandardOffsetUnits=m  TranslationROffset=0  TranslationROffsetUnits=m  TranslationThetaOffset=0  TranslationThetaOffsetUnits=deg  TranslationZOffset=0  TranslationZOffsetUnits=m
  W : PMIOPort  Side=Left
  P1 : PMIOPort  Port=2  Side=Right
  P2 : PMIOPort  Port=3  Side=Right
  P3 : PMIOPort  Port=4  Side=Right
  Crank : PMIOPort  Port=5  Side=Right
  connections:
  Transform P3/RConn1 -- P3/RConn1
  Transform P1/RConn1 -- P1/RConn1
  Transform P3/LConn1 -- Transform Shell/LConn1 -- Transform Crank Axis/LConn1 -- W/RConn1 -- P2/RConn1 -- Transform P1/LConn1
  Transform Shell/RConn1 -- Shell/LConn1
  Transform Crank Axis/RConn1 -- Bearing Fault Visual/LConn1 -- Crank/RConn1

== system sm_pump_triplex/Sensing pq Out/Compare ==
  pOut : Inport
  Measured Data : FromWorkspace  VariableName=[pOutMeas_time pOutMeas_data]  OutputAfterFinalValue=Holding final value
  Output Pressure : Scope  NumInputPorts=2
      settings: Title=Output Pressure: Compare with Measured Data  ActiveDisplayYMinimum=6.95756  ActiveDisplayYMaximum=7.33433
  Zero-Order Hold : ZeroOrderHold  SampleTime=-1
  wires:
  pOut/1 -> Output Pressure/1  "Simulation"
  Measured Data/1 -> Zero-Order Hold/1
  Zero-Order Hold/1 -> Output Pressure/2  "Measured"

== system sm_pump_triplex/Sensing pq Out/Meas Scope ==
  pMeas : Inport
  Output Pressure Measurement : Scope
      settings: TimeSpan=1  ActiveDisplayYMinimum=6.95483  ActiveDisplayYMaximum=7.36166
  wires:
  pMeas/1 -> Output Pressure Measurement/1

== system sm_pump_triplex/Diagnostics/Diagnostics/Off ==
  pOut : Inport
  Constant : Constant  OutDataTypeStr=int8
  Constant1 : Constant  Value=[1 1 1 1]*-1
  Terminator : Terminator
  fault : Outport  VectorParamsAs1DForOutWhenUnconnected=off
  hmi : Outport  Port=2  VectorParamsAs1DForOutWhenUnconnected=off
  wires:
  Constant1/1 -> hmi/1
  Constant/1 -> fault/1
  pOut/1 -> Terminator/1

== system sm_pump_triplex/Diagnostics/Diagnostics/On ==
  pOut : Inport
  Clock : Clock
  Collect Data : MATLAB Function  TreatAsAtomicUnit=on  SystemSampleTime=TRP_Par.Sensors.q.Ts
  FFT and Classification : MATLAB Function  TreatAsAtomicUnit=on  SystemSampleTime=TRP_Par.Sensors.q.Ts*100
  Motor Speed (RPM) : Constant  Value=TRP_Par.Spec.target_spd
  Steady State : simulink/Logic and Bit Operations/Compare To Constant  relop=>=  const=time_steady_state  OutDataTypeStr=boolean  ZeroCross=off
  fault : Outport  VectorParamsAs1DForOutWhenUnconnected=off
  hmi : Outport  Port=2  VectorParamsAs1DForOutWhenUnconnected=off
  wires:
  Clock/1 -> Steady State/1
  Steady State/1 -> FFT and Classification/2(enablePred)
  FFT and Classification/1(faultState) -> fault/1
  Motor Speed (RPM)/1 -> FFT and Classification/3(cmdSpeed)
  Collect Data/1(pArray) -> FFT and Classification/1(pArray)
  pOut/1 -> Collect Data/1(pOut)
  FFT and Classification/2(hmiVec) -> hmi/1

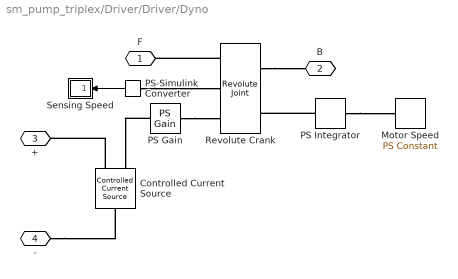
== system sm_pump_triplex/Driver/Driver/Dyno ==
  Controlled Current Source : fl_lib/Electrical/Electrical Sources/Controlled Current Source
  Motor Speed : fl_lib/Physical Signals/Sources/PS Constant  constant=TRP_Par.Spec.target_spd*2*pi/60 rad/s
  PS Gain : fl_lib/Physical Signals/Functions/PS Gain  gain=1 A/(N*m)
  PS Integrator : fl_lib/Physical Signals/Linear Operators/PS Integrator  reset_method=foundation.enum.IntegratorResetSpec.None  initial_condition_spec=foundation.enum.IntegratorICSpec.Internal  saturation_spec=foundation.enum.IntegratorSaturationSpec.None  saturation_source_spec=foundation.enum.IntegratorSaturationSourceSpec.Internal  x0=0  xu=inf s  xl=-inf s
  PS-Simulink Converter : nesl_utility/PS-Simulink Converter  PhysicalDomain=network_engine_domain  SubClassName=ps_output  LeftPortType=input  RightPortType=output  PseudoPeriodic=off  Frequencies=[]  VectorFormat=1-D array  Unit=rpm  AffineConversion=off
  Revolute Crank : sm_lib/Joints/Revolute Joint  JointMode=Normal  CompositeWrenchDir=FollowerOnBase  CompositeWrenchFrame=BaseFrame  SenseConstraintForce=off  SenseConstraintTorque=off  SenseTotalForce=off  SenseTotalTorque=off  PositionTargetSpecify=off  PositionTargetPriority=High  PositionTargetValue=0  PositionTargetValueUnits=deg  VelocityTargetSpecify=off  VelocityTargetPriority=High  VelocityTargetValue=0  VelocityTargetValueUnits=deg/s  EquilibriumPosition=0  EquilibriumPositionUnits=deg  SpringStiffness=0  SpringStiffnessUnits=N*m/deg  DampingCoefficient=0  DampingCoefficientUnits=N*m/(deg/s)  LowerLimitSpecify=off  LowerLimitBound=-90  LowerLimitBoundUnits=deg  LowerLimitStiffness=1e4  LowerLimitStiffnessUnits=N*m/deg  LowerLimitDamping=10  LowerLimitDampingUnits=N*m/(deg/s)  LowerLimitTransitionRegionWidth=0.1  LowerLimitTransitionRegionWidthUnits=deg  UpperLimitSpecify=off  UpperLimitBound=90  UpperLimitBoundUnits=deg  UpperLimitStiffness=1e4  UpperLimitStiffnessUnits=N*m/deg  UpperLimitDamping=10  UpperLimitDampingUnits=N*m/(deg/s)  UpperLimitTransitionRegionWidth=0.1  UpperLimitTransitionRegionWidthUnits=deg  TorqueActuationMode=ComputedTorque  MotionActuationMode=InputMotion  SensePosition=off  SenseVelocity=on  SenseAcceleration=off  SenseTorqueForce=on  SenseLowerLimitTorqueForce=off  SenseUpperLimitTorqueForce=off
  Sensing Speed : Subsystem
  F : PMIOPort  Side=Right
  B : PMIOPort  Port=2  Side=Right
  + : PMIOPort  Port=3  Side=Left
  - : PMIOPort  Port=4  Side=Left
  wires:
  PS-Simulink Converter/1 -> Sensing Speed/1(w)
  connections:
  -/RConn1 -- Controlled Current Source/LConn1
  Controlled Current Source/RConn2 -- +/RConn1
  Revolute Crank/LConn1 -- B/RConn1
  Revolute Crank/RConn1 -- F/RConn1
  PS Gain/RConn1 -- Controlled Current Source/RConn1
  PS Integrator/RConn1 -- Revolute Crank/LConn2
  PS Integrator/LConn1 -- Motor Speed/RConn1
  PS Gain/LConn1 -- Revolute Crank/RConn3
  PS-Simulink Converter/LConn1 -- Revolute Crank/RConn2

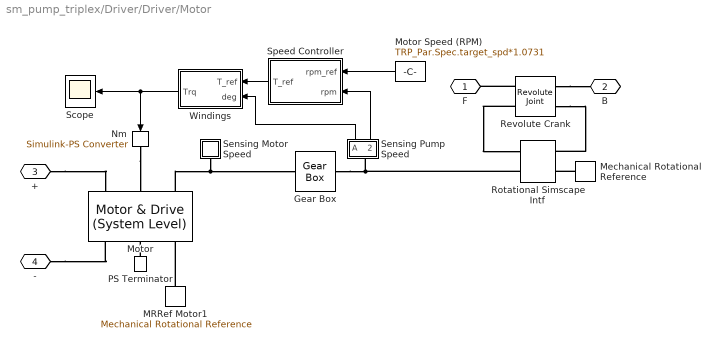
== system sm_pump_triplex/Driver/Driver/Motor ==
  Gear Box : fl_lib/Mechanical/Mechanisms/Gear Box  ratio=TRP_Par.Motor.Gear.ratio  t_in_specify=off  t_in_priority=None  t_in=0 N*m  t_in_nominal_specify=off  t_in_nominal_value=1  t_in_nominal_unit=N*m  t_out_specify=off  t_out_priority=None  t_out=0 N*m  t_out_nominal_specify=off  t_out_nominal_value=1  t_out_nominal_unit=N*m
  MRRef Motor1 : fl_lib/Mechanical/Rotational Elements/Mechanical Rotational Reference  Tag=Factory Generic
  Mechanical Rotational Reference : fl_lib/Mechanical/Rotational Elements/Mechanical Rotational Reference
  Motor : ee_lib/Electromechanical/Motor & Drive (System Level)  torque_speed_param=2  overtorque_param=ee.enum.electromech.overtorque.no  T_t=[.09, .08, .07, 0] N*m  T_t_intermittent=[.36, .32, .28, 0] N*m  T_t_2D=[.09, .09, .09; .08, .08, .08; .07, .07, .07; 0, 0, 0] N*m  T_t_intermittent_2D=[.36, .36, .36; .32, .32, .32; .28, .28, .28; 0, 0, 0] N*m  w_t=[0, 3750, 7500, 8000] rpm  vdc_t=[6, 12, 24] V  torque_max=5 N*m  power_max=9000 W  torque_max_intermittent=0.4 N*m  power_max_intermittent=120 W  time_overtorque=30 s  time_recover=60 s  Tc=0.02 s  EnableSwitch=simscape.enum.onoff.off  losses_param=1  eff=100  w_eff=958 rpm  T_eff=1 N*m  Piron=0 W  Pbase=0 W  w_eff_vec=[-8000, -4000, 0, 4000, 8000] rpm  T_eff_vec=[0, .03, .06, .09] N*m  v_eff_vec=[100, 250, 400] V  losses_mat=[1.49, 1.67, 2.21, 3.1; .42, .69, 1.14, 2.03; .06, .24, .78, 1.68; .42, .69, 1.14, 2.03; 1.49, 1.67, 2.21, 3.1] W  efficiency_mat=[95, 95, 95, 95; 95, 95, 95, 95; 95, 95, 95, 95; 95, 95, 95, 95; 95, 95, 95, 95]  losses_mat_3D=ones(5, 4, 3) W  efficiency_mat_3D=95 * ones(5, 4, 3)  Res=0 Ohm  J=5e-6*0 kg*m^2  lam=1e-5*0 N*m/(rad/s)  speed0=0 rpm  faulted_specify=off  faulted_priority=None  faulted=0  faulted_nominal_specify=off  faulted_nominal_value=1  faulted_nominal_unit=1  isSwitchedOff_specify=off  isSwitchedOff_priority=None  isSwitchedOff=0  isSwitchedOff_nominal_specify=off  isSwitchedOff_nominal_value=1  isSwitchedOff_nominal_unit=1  torqueLimitContinuous_specify=off  torqueLimitContinuous_priority=None  torqueLimitContinuous=0 N*m  torqueLimitContinuous_nominal_specify=off  torqueLimitContinuous_nominal_value=1  torqueLimitContinuous_nominal_unit=N*m  alpha=3.93e-3 1/K  Tmeas=25 degC  Tmeas2=125 degC  losses_mat_T2=[1.49, 1.74, 2.49, 3.74; .42, .67, 1.42, 2.67; .06, .31, 1.06, 2.31; .42, .67, 1.42, 2.67; 1.49, 1.74, 2.49, 3.74] W  efficiency_mat_T2=[95, 95, 95, 95; 95, 95, 95, 95; 95, 95, 95, 95; 95, 95, 95, 95; 95, 95, 95, 95]  losses_mat_3D_T2=ones(5, 4, 3) W  efficiency_mat_3D_T2=95 * ones(5, 4, 3)  thermal_mass=100 J/K  initial_temperature=25 degC
  Motor Speed (RPM) : Constant  Value=TRP_Par.Spec.target_spd*1.0731
  Nm : nesl_utility/Simulink-PS Converter  PhysicalDomain=network_engine_domain  SubClassName=ps_input  LeftPortType=input  RightPortType=output  PseudoPeriodic=off  Frequencies=[]  NoiseDistribution=none  NoiseParameters=[]  Unit=N*m  AffineConversion=off  FilteringAndDerivatives=zero  SimscapeFilterOrder=1  InputFilterTimeConstant=0.005  UdotUserProvided=1
  PS Terminator : fl_lib/Physical Signals/Sinks/PS Terminator
  Revolute Crank : sm_lib/Joints/Revolute Joint  JointMode=Normal  CompositeWrenchDir=FollowerOnBase  CompositeWrenchFrame=BaseFrame  SenseConstraintForce=off  SenseConstraintTorque=off  SenseTotalForce=off  SenseTotalTorque=off  PositionTargetSpecify=off  PositionTargetPriority=High  PositionTargetValue=0  PositionTargetValueUnits=deg  VelocityTargetSpecify=off  VelocityTargetPriority=High  VelocityTargetValue=0  VelocityTargetValueUnits=deg/s  EquilibriumPosition=0  EquilibriumPositionUnits=deg  SpringStiffness=0  SpringStiffnessUnits=N*m/deg  DampingCoefficient=0  DampingCoefficientUnits=N*m/(deg/s)  LowerLimitSpecify=off  LowerLimitBound=-90  LowerLimitBoundUnits=deg  LowerLimitStiffness=1e4  LowerLimitStiffnessUnits=N*m/deg  LowerLimitDamping=10  LowerLimitDampingUnits=N*m/(deg/s)  LowerLimitTransitionRegionWidth=0.1  LowerLimitTransitionRegionWidthUnits=deg  UpperLimitSpecify=off  UpperLimitBound=90  UpperLimitBoundUnits=deg  UpperLimitStiffness=1e4  UpperLimitStiffnessUnits=N*m/deg  UpperLimitDamping=10  UpperLimitDampingUnits=N*m/(deg/s)  UpperLimitTransitionRegionWidth=0.1  UpperLimitTransitionRegionWidthUnits=deg  TorqueActuationMode=InputTorque  MotionActuationMode=ComputedMotion  SensePosition=off  SenseVelocity=on  SenseAcceleration=off  SenseTorqueForce=off  SenseLowerLimitTorqueForce=off  SenseUpperLimitTorqueForce=off
  Rotational Simscape Intf : Multibody_Multiphysics_Lib/Interfaces/Rotational Simscape Intf  SystemSampleTime=-1  VariantActivationTime=update diagram  EmptyChoice=off  PassThrough=off  PassThroughVariantControl=(default)  EmptyChoiceVariantControl=(default)  AllowFlexibleInterface=on  Latency=0  AutoFrameSizeCalculation=off
      settings: SourceProductName=Simscape Multibody Multiphysics Library
  Scope : Scope
      settings: ActiveDisplayYMinimum=-2.40087  ActiveDisplayYMaximum=21.60781
  Sensing Motor Speed : Subsystem
      mask Display: disp('w')
  Sensing Pump Speed : Subsystem
      mask Display: disp('A,w')
  Speed Controller : Subsystem
  Windings : Subsystem
  F : PMIOPort  Side=Right
  B : PMIOPort  Port=2  Side=Right
  + : PMIOPort  Port=3  Side=Left
  - : PMIOPort  Port=4  Side=Left
  wires:
  Windings/1(Trq) -> Scope/1, Nm/1
  Sensing Pump Speed/1(A) -> Windings/2(deg)
  Motor Speed (RPM)/1 -> Speed Controller/1(rpm_ref)
  Speed Controller/1(T_ref) -> Windings/1(T_ref)
  Sensing Pump Speed/2(rpm) -> Speed Controller/2(rpm)
  connections:
  MRRef Motor1/LConn1 -- Motor/RConn3
  Revolute Crank/LConn2 -- Rotational Simscape Intf/LConn1
  Revolute Crank/RConn1 -- F/RConn1
  Sensing Pump Speed/LConn1 -- Gear Box/RConn1 -- Rotational Simscape Intf/RConn2
  Revolute Crank/LConn1 -- B/RConn1
  Mechanical Rotational Reference/LConn1 -- Rotational Simscape Intf/LConn2
  Revolute Crank/RConn2 -- Rotational Simscape Intf/RConn1
  Motor/LConn3 -- Gear Box/LConn1 -- Sensing Motor Speed/LConn1
  +/RConn1 -- Motor/LConn1
  -/RConn1 -- Motor/RConn1
  PS Terminator/LConn1 -- Motor/RConn2
  Nm/RConn1 -- Motor/LConn2
